simulink model "Copy_2_of_simulation"  (R2026b)
settings: Solver=ode23s  StopTime=T_sim  MaxStep=1e-3  MinStep=1e-7  RelTol=1e-5
InitFcn:
  | run param_file_2.m
values from neighbouring files (symbols this model uses):
  param = struct()    [param_file.m]    (also in param_file_2.m)
(part 2 of 2)

== matlab function Copy_2_of_simulation/MATLAB Function3 ==
  settings: updateMethod=DISCRETE  sampleTime=1e-5
  data: Pdes input; param parameter; PX input; open_PRV output; open_SSV output; PRV_position input; SSV_position input; omega input
% function [open_PRV, open_SSV] = fcn(Pdes, PX, param)
% 
% % Pressure margin for valve closure
% pressure_margin = 0.5e6;  % 0.5 MPa
% 
% if Pdes == param.P_H
% 
%     open_PRV = 1;
% 
%     % Only compress if below the high rail
%     if PX < param.P_H - pressure_margin
%         open_SSV = 1;
%     else
%         open_SSV = 0;
%     end
% 
% else
% 
%     open_PRV = -1;
% 
%     % Only decompress if above the medium rail
%     if PX > param.P_M + pressure_margin
%         open_SSV = -1;
%     else
%         open_SSV = 0;
%     end
% 
% end
% 
% end
function [open_PRV, open_SSV] = fcn(Pdes, param, PX, ...
    PRV_position, SSV_position, omega)

persistent phase switch_number current_rail

HOLD        = uint8(1);
CAPTURE     = uint8(2);
USE_ENERGY  = uint8(3);
SELECT_RAIL = uint8(4);

if isempty(phase)
    phase = HOLD;
    switch_number = uint8(1);
    current_rail = -1;          % Start on medium
end

pressure_tol = 1e4;             % Pa, 0.1 bar
spool_ready = 0.95;
ssv_center_band = 0.02;

% Each switch goes to the opposite rail.
target_rail = -current_rail;
if target_rail == 1
    target_pressure = param.P_H;
else
    target_pressure = param.P_M;
end

% Upward switch: ready when PX >= P_H - pressure_tol.
% Downward switch: ready when PX <= P_M + pressure_tol.
pressure_ready = target_rail * (target_pressure - PX) <= pressure_tol;
prv_ready = target_rail * PRV_position >= spool_ready;
switch_complete = false;

switch phase
    % case HOLD
    %     if switch_number <= 5 && Pdes == target_pressure && ...
    %             abs(SSV_position) <= ssv_center_band
    %         if switch_number <= 3
    %             phase = CAPTURE;
    %         else
    %             phase = USE_ENERGY;
    %         end
    %     end
    case HOLD
        if switch_number <= 3 && Pdes == target_pressure && ...
                abs(SSV_position) <= ssv_center_band
            if switch_number <= 2
                phase = CAPTURE;
            else
                phase = USE_ENERGY;
            end
        end

    case CAPTURE
        % The new rail is selected while the SSV routes flow through
        % the motor. Center the SSV once the transition is complete.
        if prv_ready && pressure_ready
            switch_complete = true;
        end

    case USE_ENERGY
        % Keep the previous rail selected while the shaft drives the pump.
        % Hand off at target pressure, or if the shaft runs out of speed.
        if pressure_ready || omega <= 0
            phase = SELECT_RAIL;
        end

    case SELECT_RAIL
        % Keep the SSV shifted while the PRV travels to the new rail.
        if prv_ready
            switch_complete = true;
        end
end

if switch_complete
    current_rail = target_rail;
    switch_number = switch_number + uint8(1);
    phase = HOLD;
end

% In HOLD, the selected rail stays connected and the SSV centers.
open_PRV = current_rail;
open_SSV = 0;

switch phase
    case {CAPTURE, SELECT_RAIL}
        open_PRV = target_rail;
        open_SSV = target_rail;

    case USE_ENERGY
        open_PRV = current_rail;
        open_SSV = target_rail;
end
end
%%
% function [open_PRV, open_SSV] = fcn(Pdes, clock_time, param)
% 
% t = clock_time(1);      % Simulation time [s]
% t_select_high = 0.244;  % Command PRV to high [s]
% t_center_SSV  = 0.251;  % Command SSV to center [s]
% 
% if Pdes ~= param.P_H
%     % Medium requested: select medium and center the SSV.
%     open_PRV = -1;
%     open_SSV =  0;
% 
% elseif t < t_select_high
%     % High requested: pump from medium into the chamber.
%     open_PRV = -1;
%     open_SSV =  1;
% 
% elseif t < t_center_SSV
%     % Select high while keeping the pump connected.
%     open_PRV =  1;
%     open_SSV =  1;
% 
% else
%     % Hold high and let the shaft coast.
%     open_PRV =  1;
%     open_SSV =  0;
% end
% 
% end
%%
% function [open_PRV, open_SSV] = fcn(Pdes, param, PX, ...
%     PRV_position, SSV_position, omega)
% 
% persistent stage
% 
% if isempty(stage)
%     stage = uint8(1);
% end
% 
% switch stage
%     case 1  % Hold medium until high is requested
%         if Pdes == param.P_H
%             stage = uint8(2);
%         end
% 
%     case 2  % Pump from medium into the chamber using shaft kinetic energy
%         if PX >= param.P_H
%             stage = uint8(3);
%         end
% 
%     case 3  % Wait until the PRV has physically moved to high
%         if PRV_position >= 0.95
%             stage = uint8(4);
%         end
% end
% 
% switch stage
%     case 1
%         open_PRV = -1;
%         open_SSV =  0;
%     case 2
%         open_PRV = -1;
%         open_SSV =  1;
%     case 3
%         open_PRV =  1;
%         open_SSV =  1;
%     otherwise  % Hold high for the rest of the run
%         open_PRV =  1;
%         open_SSV =  0;
% end
% end
%% New
% function [open_PRV, open_SSV] = fcn(Pdes, param, PX, ...
%     PRV_position, SSV_position, omega)
% % PRV: +1 = high rail, -1 = medium rail
% % SSV:  0 = direct rail-to-chamber connection
% %      +1 = rail to motor P, chamber to motor T
% %      -1 = chamber to motor P, rail to motor T
% 
% persistent stage
% 
% HOLD_MEDIUM    = uint8(1);
% CHARGE_TO_HIGH = uint8(2);
% HOLD_HIGH      = uint8(3);
% RETURN_TO_HIGH = uint8(4);
% SELECT_MEDIUM  = uint8(5);
% 
% if isempty(stage)
%     stage = HOLD_MEDIUM;
% end
% 
% medium_switch_margin = 0.1e6;  % Pa above the medium rail
% 
% pressure_tol = 1e4;   % Pa, same as the existing relay's 0.1 bar tolerance
% spool_ready  = 0.95;  % 95% of normalized PRV travel
% 
% % Advance the sequence using chamber pressure and actual valve position.
% switch stage
%     case HOLD_MEDIUM
%         if Pdes == param.P_H
%             stage = CHARGE_TO_HIGH;
%         end
% 
%     case CHARGE_TO_HIGH
%         if PX >= param.P_H - pressure_tol && PRV_position >= spool_ready
%             stage = HOLD_HIGH;
%         end
% 
%     case HOLD_HIGH
%         if Pdes == param.P_M
%             stage = RETURN_TO_HIGH;
%         end
% 
%     % case RETURN_TO_HIGH
%     %     % The shaft starts recovery spinning in the positive direction.
%     %     % At the first zero crossing, command the PRV to medium.
%     %     if omega <= 0
%     %         stage = SELECT_MEDIUM;
%     %     end
% 
%     case RETURN_TO_HIGH
%         if PX <= param.P_M + medium_switch_margin
%             stage = SELECT_MEDIUM;
%         end
% 
%     case SELECT_MEDIUM
%         % Keep the SSV shifted until the PRV has physically moved to medium.
%         if PRV_position <= -spool_ready
%             stage = HOLD_MEDIUM;
%         end
% end
% 
% % Issue the valve commands for the current stage.
% switch stage
%     case HOLD_MEDIUM
%         open_PRV = -1;
%         open_SSV =  0;
% 
%     case CHARGE_TO_HIGH
%         open_PRV =  1;
%         open_SSV =  1;
% 
%     case HOLD_HIGH
%         open_PRV =  1;
%         open_SSV =  0;
% 
%     case RETURN_TO_HIGH
%         open_PRV =  1;
%         open_SSV = -1;
% 
%     case SELECT_MEDIUM
%         open_PRV = -1;
%         open_SSV = -1;
% 
%     otherwise
%         open_PRV = -1;
%         open_SSV =  0;
% end
% end

%% Old
% function [open_PRV, open_SSV] = fcn(Pdes, param, PX, ...
%     PRV_position, SSV_position, omega)
% 
% persistent stage
% 
% HOLD_MEDIUM         = uint8(1);
% CHARGE_TO_HIGH      = uint8(2);
% HOLD_HIGH           = uint8(3);
% DISCHARGE_TO_MEDIUM = uint8(4);
% 
% if isempty(stage)
%     stage = HOLD_MEDIUM;
% end
% 
% pressure_tol = 1e4;   % Pa (0.1 bar)
% spool_ready  = 0.95;  % 95% of normalized PRV travel
% 
% % Advance the switching sequence.
% switch stage
%     case HOLD_MEDIUM
%         if Pdes == param.P_H
%             stage = CHARGE_TO_HIGH;
%         end
% 
%     case CHARGE_TO_HIGH
%         if PX >= param.P_H - pressure_tol && PRV_position >= spool_ready
%             stage = HOLD_HIGH;
%         end
% 
%     case HOLD_HIGH
%         if Pdes == param.P_M
%             stage = DISCHARGE_TO_MEDIUM;
%         end
% 
%     case DISCHARGE_TO_MEDIUM
%         if abs(PX - param.P_M) <= pressure_tol && ...
%                 PRV_position <= -spool_ready
%             stage = HOLD_MEDIUM;
%         end
% end
% 
% % Set valve commands for the current stage.
% switch stage
%     case CHARGE_TO_HIGH
%         open_PRV =  1;
%         open_SSV =  1;
% 
%     case HOLD_HIGH
%         open_PRV =  1;
%         open_SSV =  0;
% 
%     case DISCHARGE_TO_MEDIUM
%         open_PRV = -1;
%         open_SSV = -1;
% 
%     otherwise  % HOLD_MEDIUM
%         open_PRV = -1;
%         open_SSV =  0;
% end
% end

%% Super new
% function [open_PRV, open_SSV] = fcn(Pdes, param, PX, ...
%     PRV_position, SSV_position, omega)
% 
% persistent phase switch_number current_rail
% 
% HOLD        = uint8(1);
% STORE       = uint8(2);
% USE_ENERGY  = uint8(3);
% SELECT_RAIL = uint8(4);
% 
% if isempty(phase)
%     phase = HOLD;
%     switch_number = uint8(1);   % Next switch in the four-switch cycle
%     current_rail = -1;          % Start on medium
% end
% 
% pressure_tol    = 1e4;    % Pa, for completing a storage switch
% spool_ready     = 0.95;
% ssv_center_band = 0.02;
% 
% recovery_margin = 0.4e6;  % Switch 3: hand off 0.4 MPa below high
% P_switch4       = 4.9e6;  % Switch 4: command medium as PX falls to 5.1 MPa
% 
% % The requested sequence alternates between the two rails.
% target_rail = -current_rail;
% if target_rail == 1
%     target_pressure = param.P_H;
% else
%     target_pressure = param.P_M;
% end
% 
% % Positive while the chamber still has pressure left to gain or lose.
% pressure_remaining = target_rail * (target_pressure - PX);
% prv_at_target = target_rail * PRV_position >= spool_ready;
% 
% switch phase
%     case HOLD
%         if Pdes == target_pressure && abs(SSV_position) <= ssv_center_band
%             if switch_number <= 2
%                 phase = STORE;
%             else
%                 phase = USE_ENERGY;
%             end
%         end
% 
%     case STORE
%         % Switches 1 and 2: the pressure difference drives the shaft.
%         if prv_at_target && pressure_remaining <= pressure_tol
%             phase = HOLD;
%         end
% 
%     case USE_ENERGY
%         if switch_number == 4
%             pressure_ready = PX <= P_switch4;
%         else
%             pressure_ready = pressure_remaining <= recovery_margin;
%         end
% 
%         if pressure_ready || omega <= 0
%             phase = SELECT_RAIL;
%         end
% 
%     case SELECT_RAIL
%         % Keep the SSV shifted until the PRV reaches the target rail.
%         if prv_at_target
%             phase = HOLD;
%         end
% end
% 
% % Count a completed switch only after the PRV reaches the new rail.
% if phase == HOLD && prv_at_target
%     current_rail = target_rail;
%     if switch_number == 4
%         switch_number = uint8(1);
%     else
%         switch_number = switch_number + uint8(1);
%     end
% end
% 
% % In HOLD, center the SSV so the shaft can coast between switches.
% open_PRV = current_rail;
% open_SSV = 0;
% 
% switch phase
%     case {STORE, SELECT_RAIL}
%         open_PRV = target_rail;
%         open_SSV = target_rail;
% 
%     case USE_ENERGY
%         open_PRV = current_rail;
%         open_SSV = target_rail;
% end
% end

%% Super super new
    % function [open_PRV, open_SSV] = fcn(Pdes, param, PX, ...
    %         PRV_position, SSV_position, omega)
    % 
    %     persistent phase switch_number current_rail
    % 
    %     HOLD        = uint8(3);
    %     STORE       = uint8(4);
    %     USE_ENERGY  = uint8(2);
    %     SELECT_RAIL = uint8(1);
    % 
    %     if isempty(phase)
    %         phase = HOLD;
    %         switch_number = uint8(1);   % Next switch in the five-switch cycle
    %         current_rail = -1;          % Start on the medium rail
    %     end
    % 
    %     pressure_tol      = 1e4;    % Pa, storage-switch completion tolerance
    %     spool_ready       = 0.95;   % PRV is within 5% of its target position
    %     ssv_center_band   = 0.02;   % SSV center deadband
    %     recovery_margin   = 0.5e6;  % Pa below high for upward recovery
    %     P_handoff_down    = 4.9e6;  % Pa, chamber pressure for downward recovery
    % 
    %     % Rail positions: +1 = high, -1 = medium.
    %     target_rail = -current_rail;
    %     if target_rail == 1
    %         target_pressure = param.P_H;
    %     else
    %         target_pressure = param.P_M;
    %     end
    % 
    %     % Positive until chamber pressure reaches the target in either direction.
    %     pressure_remaining = target_rail * (target_pressure - PX);
    %     prv_at_target = target_rail * PRV_position >= spool_ready;
    % 
    %     switch_complete = false;
    % 
    %     switch phase
    %         case HOLD
    %             if Pdes == target_pressure && abs(SSV_position) <= ssv_center_band
    %                 if switch_number <= 3
    %                     phase = STORE;
    %                 else
    %                     phase = USE_ENERGY;
    %                 end
    %             end
    % 
    %         case STORE
    %             % Switches 1-3: select the target rail and accelerate the shaft.
    %             if prv_at_target && pressure_remaining <= pressure_tol
    %                 switch_complete = true;
    %             end
    % 
    %         case USE_ENERGY
    %             % Switches 4-5: keep the starting rail selected while pumping.
    %             if target_rail == -1
    %                 % High to medium: pump chamber oil back into the high rail.
    %                 pressure_ready = PX <= P_handoff_down;
    %             else
    %                 % Medium to high: pump oil from medium into the chamber.
    %                 pressure_ready = PX >= param.P_H - recovery_margin;
    %             end
    % 
    %             if pressure_ready || omega <= 0
    %                 phase = SELECT_RAIL;
    %             end
    % 
    %         case SELECT_RAIL
    %             % Keep the SSV shifted until the PRV reaches the target rail.
    %             if prv_at_target
    %                 switch_complete = true;
    %             end
    %     end
    % 
    %     % Count each completed switch once, then command the SSV to center.
    %     if switch_complete
    %         current_rail = target_rail;
    %         phase = HOLD;
    % 
    %         if switch_number == 5
    %             switch_number = uint8(1);
    %         else
    %             switch_number = switch_number + uint8(1);
    %         end
    %     end
    % 
    %     % Default HOLD commands: stay on the selected rail and coast.
    %     open_PRV = current_rail;
    %     open_SSV = 0;
    % 
    %     switch phase
    %         case {STORE, SELECT_RAIL}
    %             open_PRV = target_rail;
    %             open_SSV = target_rail;
    % 
    %         case USE_ENERGY
    %             open_PRV = current_rail;
    %             open_SSV = target_rail;
    %     end
    % 
    % end

== matlab function Copy_2_of_simulation/MATLAB Function9 ==
  data: P input; P_initial input; Win output; param parameter
function Win = oil_comp(P,P_initial,param)

Pg = P-param.P_T;   % Gauge pressure
r = P/param.P_T;    % Pressure ratio
e = exp(Pg/param.beta); 
rv = (1./e+param.air*r.^(-1/param.gamma))/(1+param.air);      %Volume ratio

El = param.beta*(e - (1 + Pg/param.beta)) + param.P_T*(e - 1);              % Energy in liquid
Eg = P/(param.gamma - 1) .* (1 - r.^(1/param.gamma - 1));           % Energy in gas
E  = (El./e + param.air*Eg.*r.^(-1/param.gamma)) ./ ...
     (1./e + param.air*r.^(-1/param.gamma));                       % Energy in mixture
Win  = E - (1./rv - 1)*P_initial;                                 % Compressibility energy density

== matlab function Copy_2_of_simulation/MATLAB Function1 ==
  data: current input; omega input; Tau_Elec output; param parameter; Tau_Mech output; Tau_Elec_Fric output
function [Tau_Elec, Tau_Mech, Tau_Elec_Fric] = BLDC(current, omega, param)

% Limit current to stall current
I_stall = 69;
current = min(max(current, -I_stall), I_stall);

% Electromagnetic torque
Tau_Elec = param.Kt * current;

% Friction torque (viscous model)
Tau_Elec_Fric = param.B * omega;

% Mechanical torque available at shaft
Tau_Mech = Tau_Elec - Tau_Elec_Fric;

end

== matlab function Copy_2_of_simulation/MATLAB Function2 ==
  data: Ph1 input; PA input; Qh1 input; Qh1dot output; param parameter
function Qh1dot = Small_Vol_A_Hose_Dynamics(Ph1, PA, Qh1, param)

Qh1dot = ((Ph1 - PA) - param.ResistHose*Qh1)/param.InertHose;

== matlab function Copy_2_of_simulation/Electric Torque Controller1 ==
  data: Control_Signal input; Kp input; omega input; T_elec output; start_final_velocity input; T_elec_max input; param parameter
% function T_elec  = fcn(Control_Signal, Kp, omega, start_final_velocity, T_elec_max, param)
% 
% if Control_Signal == 1 
% 
%     if omega < start_final_velocity
%         omega_error = omega -start_final_velocity;
%         T_elec = - (Kp*omega_error);
%     else
%         T_elec = -T_elec_max;
%     end
% 
% else
%     if omega >= param.max_speed-0.01
%         omega_error = omega - param.max_speed;
%         T_elec = -(Kp*omega_error);
%     else
%         T_elec = T_elec_max;
%     end
% 
% end

function T_elec = fcn(Control_Signal, Kp, omega, ...
    start_final_velocity, T_elec_max, param)

if Control_Signal == 1
    target_speed = start_final_velocity;
else
    target_speed = param.max_speed;
end

omega_error = omega - target_speed;

T_elec = -Kp * omega_error;

% Saturate torque
T_elec = min(max(T_elec, -T_elec_max), T_elec_max);

end

== matlab function Copy_2_of_simulation/Small Volume A1 ==
  data: Qh1 input; QA input; PAdot output; param parameter
function PAdot = Small_Vol_A(Qh1,QA, param)

PAdot = (param.beta/param.VA_0)*(Qh1-QA);

== matlab function Copy_2_of_simulation/MATLAB Function4 ==
  data: Ph1 input; PA input; Qh1 output; param parameter
function Qh1 = Small_Vol_A_Hose_Dynamics(Ph1, PA, param)

Qh1 = (Ph1 - PA)/param.ResistHose;

== matlab function Copy_2_of_simulation/Small Volume A2 ==
  data: Q1 input; PAdot output; QA input; beta_mix input; param parameter
function PAdot = Small_Vol_A(Q1,QA, beta_mix, param)

PAdot = (beta_mix/param.VA_0)*(Q1-QA);

== matlab function Copy_2_of_simulation/MATLAB Function5 ==
  data: P input; P_initial input; beta_mix_A output; param parameter; WA output
function [beta_mix_A, WA] = oil_comp(P,P_initial,param)

Pg = P-param.P_T;   % Gauge pressure
r = P/param.P_T;    % Pressure ratio
e = exp(Pg/param.beta); 
rv = (1./e+param.air*r.^(-1/param.gamma))/(1+param.air);      %Volume ratio

beta_mix_A = rv*(1+param.air)/(1/(e*param.beta)+...
           param.air/(param.gamma*param.P_T*r^(1/param.gamma+1)));

El = param.beta*(e - (1 + Pg/param.beta)) + param.P_T*(e - 1);              % Energy in liquid
Eg = P/(param.gamma - 1) .* (1 - r.^(1/param.gamma - 1));           % Energy in gas
E  = (El./e + param.air*Eg.*r.^(-1/param.gamma)) ./ ...
     (1./e + param.air*r.^(-1/param.gamma));                       % Energy in mixture
WA  = E - (1./rv - 1)*P_initial;                                 % Compressibility energy density

== matlab function Copy_2_of_simulation/MATLAB Function6 ==
  data: P input; P_initial input; beta_mix output; param parameter; WP output
function [beta_mix, WP] = oil_comp(P,P_initial,param)

%Ph=7e6, P0=1e5
Pg = P-param.P_T;   % Gauge pressure
r = P/param.P_T;    % Pressure ratio
e = exp(Pg/param.beta); 
rv = (1./e+param.air*r.^(-1/param.gamma))/(1+param.air);      %Volume ratio

beta_mix = rv*(1+param.air)/(1/(e*param.beta)+...
           param.air/(param.gamma*param.P_T*r^(1/param.gamma+1)));

El = param.beta*(e - (1 + Pg/param.beta)) + param.P_T*(e - 1);              % Energy in liquid
Eg = P/(param.gamma - 1) .* (1 - r.^(1/param.gamma - 1));           % Energy in gas
E  = (El./e + param.air*Eg.*r.^(-1/param.gamma)) ./ ...
     (1./e + param.air*r.^(-1/param.gamma));                       % Energy in mixture
WP  = E - (1./rv - 1)*P_initial;                                 % Compressibility energy density

== matlab function Copy_2_of_simulation/Small Volume A ==
  data: Q1 input; Ph1dot output; Qh1 input; param parameter
function Ph1dot = Small_Vol_A(Q1,Qh1, param)

Ph1dot = (param.beta/param.VA_0)*(Q1-Qh1);

== matlab function Copy_2_of_simulation/MATLAB Function7 ==
  data: P input; P_initial input; beta_mix output; param parameter; WT output
function [beta_mix, WT] = oil_comp(P,P_initial,param)

%Ph=7e6, P0=1e5
Pg = P-param.P_T;   % Gauge pressure
r = P/param.P_T;    % Pressure ratio
e = exp(Pg/param.beta); 
rv = (1./e+param.air*r.^(-1/param.gamma))/(1+param.air);      %Volume ratio

beta_mix = rv*(1+param.air)/(1/(e*param.beta)+...
           param.air/(param.gamma*param.P_T*r^(1/param.gamma+1)));


El = param.beta*(e - (1 + Pg/param.beta)) + param.P_T*(e - 1);              % Energy in liquid
Eg = P/(param.gamma - 1) .* (1 - r.^(1/param.gamma - 1));           % Energy in gas
E  = (El./e + param.air*Eg.*r.^(-1/param.gamma)) ./ ...
     (1./e + param.air*r.^(-1/param.gamma));                       % Energy in mixture
WT  = E - (1./rv - 1)*P_initial;                                 % Compressibility energy density

== matlab function Copy_2_of_simulation/MATLAB Function8 ==
  data: P input; P_initial input; beta_mix output; param parameter; WX output
function [beta_mix, WX] = oil_comp(P,P_initial,param)

%Ph=7e6, P0=1e5
Pg = P-param.P_T;   % Gauge pressure
r = P/param.P_T;    % Pressure ratio
e = exp(Pg/param.beta); 
rv = (1./e+param.air*r.^(-1/param.gamma))/(1+param.air);      %Volume ratio

beta_mix = rv*(1+param.air)/(1/(e*param.beta)+...
           param.air/(param.gamma*param.P_T*r^(1/param.gamma+1)));

El = param.beta*(e - (1 + Pg/param.beta)) + param.P_T*(e - 1);              % Energy in liquid
Eg = P/(param.gamma - 1) .* (1 - r.^(1/param.gamma - 1));           % Energy in gas
E  = (El./e + param.air*Eg.*r.^(-1/param.gamma)) ./ ...
     (1./e + param.air*r.^(-1/param.gamma));                       % Energy in mixture
WX  = E - (1./rv - 1)*P_initial;                                 % Compressibility energy density

== matlab function Copy_2_of_simulation/MATLAB Function ==
  data: beta_mix input; Stored_Power output; Pdot input; P input; Volume input
function Stored_Power = fcn(beta_mix, Pdot, P, Volume)

Stored_Power = P*(Volume/beta_mix)*Pdot;

== matlab function Copy_2_of_simulation/MATLAB Function10 ==
  data: beta_mix input; Stored_Power output; Pdot input; P input; Volume input
function Stored_Power = fcn(beta_mix, Pdot, P, Volume)

Stored_Power = P*(Volume/beta_mix)*Pdot;

== matlab function Copy_2_of_simulation/MATLAB Function11 ==
  data: beta_mix input; Stored_Power output; Pdot input; P input; Volume input
function Stored_Power = fcn(beta_mix, Pdot, P, Volume)

Stored_Power = P*(Volume/beta_mix)*Pdot;

== matlab function Copy_2_of_simulation/MATLAB Function12 ==
  data: clock_time input; Pdes output; param parameter
function Pdes = fcn(clock_time, param)

t = clock_time(1);

if t < 0.20
    Pdes = param.P_M;
elseif t < 0.75
    Pdes = param.P_H;   % Switch 1: medium to high
elseif t < 1.30
    Pdes = param.P_M;   % Switch 2: high to medium
else
    Pdes = param.P_H;   % Switch 3: medium to high
end

end

% function Pdes = fcn(clock_time, param)
% 
% t = clock_time(1);
% 
% if (t >= 0.20 && t < 0.75) || ...
%         (t >= 1.30 && t < 1.85) || ...
%         t >= 2.40
%     Pdes = param.P_H;
% else
%     Pdes = param.P_M;
% end
% 
% end

% t = clock_time(1);
% 
% if (t >= 0.20 && t < 0.75) || ...
%         (t >= 1.30 && t < 1.85) || ...
%         t >= 2.40
%     Pdes = param.P_H;
% else
%     Pdes = param.P_M;
% end
% 
% end

% function Pdes = fcn(clock_time, param)
% 
% if (clock_time >= 0.20 && clock_time < 0.75) || ...
%         (clock_time >= 1.30 && clock_time < 1.85)
%     Pdes = param.P_H;
% else
%     Pdes = param.P_M;
% end
% 
% end

== matlab function Copy_2_of_simulation/Experimental Friction Model ==
  data: pressure input; friction output; speed input
function friction  = friction_model(pressure, speed)

C = [-2.7371712380878151e-20 -1.012140531055926e-17 1.362680380791501e-14 2.5017160289203132e-12;
    7.8175012770957013e-17 6.5819426994446848e-14 -5.7218700361030071e-11 -2.6554187394929447e-08;
    -3.0602563559828119e-14 -2.3014653747973892e-10 2.0537443634696756e-07 0.00011211247665566631;
    8.9217552784699898e-12 5.982060290372595e-08 7.3192331395694632e-05 0.083988065486528374];

p = [pressure^3; pressure^2; pressure; 1];
w = [speed^3; speed^2; speed; 1];

friction = sum((C * p) .* w);
end

== matlab function Copy_2_of_simulation/MATLAB Function13 ==
  data: current_in input; current output; elec_motor input
function current = fcn(current_in, elec_motor)

if elec_motor == 1
    current = current_in;
elseif elec_motor == 0
    current = 0;
else
    current = 0;
end

== matlab function Copy_2_of_simulation/MATLAB Function14 ==
  data: inertia output; elec_motor input; param parameter
function inertia = fcn(elec_motor, param)

if elec_motor == 1
    inertia = (param.J_hyd+param.J_elec);
elseif elec_motor == 0
    inertia = param.J_hyd;
else
    inertia = 0;
end

== matlab function Copy_2_of_simulation/MATLAB Function15 ==
  data: Q_PA input; Q_AT input; rail_power output; PA input; PRV_loss_power output; param parameter
% function [rail_power, PRV_loss_power] = fcn(Q1, PA, PRV_position, param)
% 
% if PRV_position < -param.valve_buffer
%     P_rail = param.P_M;
% elseif PRV_position > param.valve_buffer
%     P_rail = param.P_H;
% else
%     % Both rail passages are closed.
%     rail_power = 0;
%     PRV_loss_power = 0;
%     return
% end
% 
% rail_power     = P_rail * Q1;         % Signed power supplied by the rail [W]
% PRV_loss_power = (P_rail - PA) * Q1;  % Power dissipated across the PRV [W]
% end

function [rail_power, PRV_loss_power] = fcn(Q_PA, Q_AT, PA, param)

% Both flows are positive from their respective rail toward port A.
rail_power = param.P_H * Q_PA + param.P_M * Q_AT;

PRV_loss_power = (param.P_H - PA) * Q_PA + ...
    (param.P_M - PA) * Q_AT;
end

== matlab function Copy_2_of_simulation/Pressure Rail Valve ==
  data: P input; T input; Q_PA output; Q_AT output; PA input; spool_position input; param parameter
% function [Q_PA, Q_AT] = RailValve(P, T, PA, spool_position, param)
% 
% db = param.valve_buffer;
% 
% spool_position = max(-1, min(1, spool_position));
% 
% if abs(spool_position) <= db
%     f = 0;
% else
%     f = (abs(spool_position) - db) / (1 - db);
%     f = max(0, min(1, f));
% end
% 
% A_PA = 0;
% A_AT = 0;
% 
% if spool_position > db
%     A_PA = param.max_Avt * f;
% elseif spool_position < -db
%     A_AT = param.max_Avt * f;
% end
% 
% Q_PA = param.Cd * A_PA * sqrt(2/param.rho) * sqrt(abs(P-PA)) * sign(P-PA);
% Q_AT = param.Cd * A_AT * sqrt(2/param.rho) * sqrt(abs(PA-T)) * sign(T-PA);
% 
% end

function [Q_PA, Q_AT] = RailValve(P, T, PA, spool_position, param)

db = param.valve_buffer;
dp_smooth = param.dp_smooth;   % Pa: smoothing scale (0.01 bar)

spool_position = max(-1, min(1, spool_position));

if abs(spool_position) <= db
    f = 0;
else
    f = (abs(spool_position) - db) / (1 - db);
    f = max(0, min(1, f));
end

A_PA = 0;
A_AT = 0;

if spool_position > db
    A_PA = param.max_Avt * f;
elseif spool_position < -db
    A_AT = param.max_Avt * f;
end

% Positive flow is from each rail toward port A.
dP_PA = P - PA;
dP_AT = T - PA;

% Smoothed signed square-root pressure relationship.
Q_PA = param.Cd * A_PA * sqrt(2/param.rho) * ...
    dP_PA / (dP_PA^2 + dp_smooth^2)^0.25;

Q_AT = param.Cd * A_AT * sqrt(2/param.rho) * ...
    dP_AT / (dP_AT^2 + dp_smooth^2)^0.25;

end

== matlab function Copy_2_of_simulation/Electric Torque Controller2 ==
  data: Control_Signal input; Kp input; omega input; T_elec output; start_final_velocity input; T_elec_max input; param parameter
% function T_elec  = fcn(Control_Signal, Kp, omega, start_final_velocity, T_elec_max, param)
% 
% if Control_Signal == 1 
% 
%     if omega < start_final_velocity
%         omega_error = omega -start_final_velocity;
%         T_elec = - (Kp*omega_error);
%     else
%         T_elec = -T_elec_max;
%     end
% 
% else
%     if omega >= param.max_speed-0.01
%         omega_error = omega - param.max_speed;
%         T_elec = -(Kp*omega_error);
%     else
%         T_elec = T_elec_max;
%     end
% 
% end

function T_elec = fcn(Control_Signal, Kp, omega, ...
    start_final_velocity, T_elec_max, param)

if Control_Signal == 1
    target_speed = start_final_velocity;
else
    target_speed = param.max_speed;
end

omega_error = omega - target_speed;

T_elec = -Kp * omega_error;

% Saturate torque
T_elec = min(max(T_elec, -T_elec_max), T_elec_max);

end

== matlab function Copy_2_of_simulation/MATLAB Function16 ==
  data: clock_time input; Pdes output; param parameter
function Pdes = fcn(clock_time, param)

if clock_time > 0.2 && clock_time < 0.75
    Pdes = param.P_H;
else
    Pdes = param.P_M;
end

== matlab function Copy_2_of_simulation/MATLAB Function17 ==
  data: Pdes input; PX input; open_PRV output; open_SSV output; param parameter
% function [open_PRV, open_SSV] = fcn(Pdes, param, Control_signal)
% 
% if Pdes == param.P_H && Control_signal == 0
%     open_PRV = 1;
%     open_SSV = 1;
% 
% elseif Pdes == param.P_M && Control_signal == 0
%     open_PRV = -1;
%     open_SSV = -1;
% 
% elseif Pdes == param.P_H && Control_signal > 0
%     open_PRV = 1;
%     open_SSV = 0;
% 
% elseif Pdes == param.P_M && Control_signal > 0
%     open_PRV = -1;
%     open_SSV = 0;
% 
% else
%     open_PRV = 0;
%     open_SSV = 0;
% end


function [open_PRV, open_SSV] = fcn(Pdes, PX, param)

% Pressure margin for valve closure
pressure_margin = 0.5e6;  % 0.5 MPa

if Pdes == param.P_H

    open_PRV = 1;

    % Only compress if below the high rail
    if PX < param.P_H - pressure_margin
        open_SSV = 1;
    else
        open_SSV = 0;
    end

else

    open_PRV = -1;

    % Only decompress if above the medium rail
    if PX > param.P_M + pressure_margin
        open_SSV = -1;
    else
        open_SSV = 0;
    end

end

end

== matlab function Copy_2_of_simulation/Soft-switch Valve ==
  data: spool_position input; Q_P output; PP input; PA input; PB input; PT input; Q_A output; Q_B output; Q_T output; param parameter; SSV_Power_throttle output; WA input; WP input; WB input; WT input; SSV_Power_throttle_HE output
% function [Q_P, Q_A, Q_B, Q_T, SSV_Power_throttle, SSV_Power_throttle_HE] = SSV(spool_position, PP, PA, PB, PT, param, WA, WP, WB, WT)
% 
% db = 0.02; % spool deadband around zero (fraction of full stroke)
% 
% spool_position = max(-1, min(1, spool_position));
% 
% if abs(spool_position) <= db
%     f = 0;
% else
%     f = (abs(spool_position) - db) / (1 - db);
%     f = max(0, min(1, f));
% end
% 
% A_PA = 0; A_PB = 0; A_AT = 0; A_BT = 0; A_PT = 0; A_AB = 0;
% 
% if abs(spool_position) <= db
%     A_PT = param.max_Avt;
%     A_AB = param.max_Avt;
% elseif spool_position > 0
%     A_PA = param.max_Avt * f;
%     A_BT = param.max_Avt * f;
% elseif spool_position < 0
%     A_PB = param.max_Avt * f;
%     A_AT = param.max_Avt * f;
% end
% 
% Q_PA = param.Cd*A_PA*sign(PP-PA)*sqrt((2/param.rho)*abs(PP-PA));
% Q_PB = param.Cd*A_PB*sign(PP-PB)*sqrt((2/param.rho)*abs(PP-PB));
% Q_AT = param.Cd*A_AT*sign(PA-PT)*sqrt((2/param.rho)*abs(PA-PT));
% Q_BT = param.Cd*A_BT*sign(PB-PT)*sqrt((2/param.rho)*abs(PB-PT));
% Q_PT = param.Cd*A_PT*sign(PP-PT)*sqrt((2/param.rho)*abs(PP-PT));
% Q_AB = param.Cd*A_AB*sign(PA-PB)*sqrt((2/param.rho)*abs(PA-PB));
% 
% Q_P = -(Q_PA + Q_PB + Q_PT);
% Q_A =  Q_AT + Q_AB - Q_PA;
% Q_B =  Q_BT - Q_AB - Q_PB;
% Q_T =  -Q_PT - Q_AT - Q_BT;
% 
% Q_B = -Q_B;
% 
% PPg = PP - param.P_T;
% PAg = PA - param.P_T;
% PBg = PB - param.P_T;
% PTg = PT - param.P_T;
% 
% SSV_Power_throttle_HE = ...
%     abs(Q_PA)*abs((WP+PPg)-(WA+PAg)) + ...
%     abs(Q_PB)*abs((WP+PPg)-(WB+PBg)) + ...
%     abs(Q_AT)*abs((WA+PAg)-(WT+PTg)) + ...
%     abs(Q_BT)*abs((WB+PBg)-(WT+PTg)) + ...
%     abs(Q_PT)*abs((WP+PPg)-(WT+PTg)) + ...
%     abs(Q_AB)*abs((WA+PAg)-(WB+PBg));
% 
% SSV_Power_throttle = ...
%     abs(Q_PA)*abs(PP-PA) + ...
%     abs(Q_PB)*abs(PP-PB) + ...
%     abs(Q_AT)*abs(PA-PT) + ...
%     abs(Q_BT)*abs(PB-PT) + ...
%     abs(Q_PT)*abs(PP-PT) + ...
%     abs(Q_AB)*abs(PA-PB);
% 
% end

function [Q_P, Q_A, Q_B, Q_T, SSV_Power_throttle, ...
    SSV_Power_throttle_HE] = SSV(spool_position, ...
    PP, PA, PB, PT, param, WA, WP, WB, WT)

db = 0.02;        % Spool deadband
dp_smooth = param.dp_smooth;  % Pa: smoothing scale (0.01 bar)

spool_position = max(-1, min(1, spool_position));

if abs(spool_position) <= db
    f = 0;
else
    f = (abs(spool_position) - db) / (1 - db);
    f = max(0, min(1, f));
end

A_PA = 0;
A_PB = 0;
A_AT = 0;
A_BT = 0;
A_PT = 0;
A_AB = 0;

if abs(spool_position) <= db
    A_PT = param.max_Avt;
    A_AB = param.max_Avt;
elseif spool_position > 0
    A_PA = param.max_Avt * f;
    A_BT = param.max_Avt * f;
elseif spool_position < 0
    A_PB = param.max_Avt * f;
    A_AT = param.max_Avt * f;
end

% Signed pressure differences
dP_PA = PP - PA;
dP_PB = PP - PB;
dP_AT = PA - PT;
dP_BT = PB - PT;
dP_PT = PP - PT;
dP_AB = PA - PB;

% Smoothed orifice flows
C = param.Cd * sqrt(2/param.rho);

Q_PA = C*A_PA*dP_PA / (dP_PA^2 + dp_smooth^2)^0.25;
Q_PB = C*A_PB*dP_PB / (dP_PB^2 + dp_smooth^2)^0.25;
Q_AT = C*A_AT*dP_AT / (dP_AT^2 + dp_smooth^2)^0.25;
Q_BT = C*A_BT*dP_BT / (dP_BT^2 + dp_smooth^2)^0.25;
Q_PT = C*A_PT*dP_PT / (dP_PT^2 + dp_smooth^2)^0.25;
Q_AB = C*A_AB*dP_AB / (dP_AB^2 + dp_smooth^2)^0.25;

% Port flows: retain existing sign conventions
Q_P = -(Q_PA + Q_PB + Q_PT);
Q_A =  Q_AT + Q_AB - Q_PA;
Q_B =  Q_BT - Q_AB - Q_PB;
Q_T = -Q_PT - Q_AT - Q_BT;

Q_B = -Q_B;

% Gauge pressures
PPg = PP - param.P_T;
PAg = PA - param.P_T;
PBg = PB - param.P_T;
PTg = PT - param.P_T;

% Hydraulic-effort calculation: retain existing definition
SSV_Power_throttle_HE = ...
    abs(Q_PA)*abs((WP+PPg)-(WA+PAg)) + ...
    abs(Q_PB)*abs((WP+PPg)-(WB+PBg)) + ...
    abs(Q_AT)*abs((WA+PAg)-(WT+PTg)) + ...
    abs(Q_BT)*abs((WB+PBg)-(WT+PTg)) + ...
    abs(Q_PT)*abs((WP+PPg)-(WT+PTg)) + ...
    abs(Q_AB)*abs((WA+PAg)-(WB+PBg));

% Throttling power calculated using the smoothed flows
SSV_Power_throttle = ...
    abs(Q_PA)*abs(dP_PA) + ...
    abs(Q_PB)*abs(dP_PB) + ...
    abs(Q_AT)*abs(dP_AT) + ...
    abs(Q_BT)*abs(dP_BT) + ...
    abs(Q_PT)*abs(dP_PT) + ...
    abs(Q_AB)*abs(dP_AB);

end

== matlab function Copy_2_of_simulation/Small Volume P ==
  data: QP input; PPdot output; Qpump input; param parameter; beta_mix input
function PPdot = Small_Vol_P(QP,Qpump, param, beta_mix)

PPdot = (beta_mix/param.VP_0)*(QP-Qpump);

== matlab function Copy_2_of_simulation/Hydraulic Motor ==
  data: Qpump output; Qleak output; omega input; PT input; PP input; fric input; param parameter; DeltaP output; Tau_Pump output; Tau_Fric output
function [Qpump, Qleak, DeltaP, Tau_Pump, Tau_Fric] = Hyd_Motor(omega, PT, PP, fric, param)

    DeltaP = PP - PT;

    Tau_Ideal = (param.D/(2*pi)) * DeltaP;
    
    % Pump friction model
    if fric == 1
        Tau_fr_nom = ((1 - param.eta_m_nom)/param.eta_m_nom) ...
                      * (param.D/(2*pi)) * param.dp_nom;
        
        k = (Tau_fr_nom - param.tau0) / param.dp_nom;
        
        omega_nom_rad = 2*pi*param.omega_nom/60;
        
        s = tanh(4*omega/(5e-5*omega_nom_rad));
        
        Tau_Fric = (param.tau0 + k*abs(DeltaP)) * s;
    else
        Tau_Fric = 0;
    end

    Tau_Pump = Tau_Ideal - Tau_Fric;

    % Analytical leakage model (Simscape-equivalent)
    
    % Parameters
    D     = param.D;          
    eta_v = param.eta_v_nom;  % nominal volumetric efficiency
    omega_nom = param.omega_nom;      % [rad/s]
    DeltaP_nom = param.dp_nom;    % [Pa]
    rho   = param.rho;        % [kg/m^3]
    
    % Hagen–Poiseuille coefficient
    K = (D/(2*pi))*omega_nom*(1 - eta_v)/DeltaP_nom;
    
    % Mass leakage flow
    m_dot_leak = K * rho * DeltaP;
    
    % Convert to volumetric leakage
    Qleak = m_dot_leak / rho;
    
    % Ideal displacement flow
    Qideal = (D/(2*pi)) * omega;
    
    % Net flow (same convention as Simscape)
    Qpump = Qideal + Qleak;
end

== matlab function Copy_2_of_simulation/Small Volume T ==
  data: QT input; PTdot output; Qpump input; param parameter; beta_mix input
function PTdot = Small_Vol_T(QT,Qpump,param, beta_mix)

PTdot = (beta_mix/param.VT_0)*(Qpump-QT);

== matlab function Copy_2_of_simulation/Main Chamber ==
  data: QB input; PXdot output; param parameter; beta_mix input
function PXdot = Main_Chamber(QB, param, beta_mix)

PXdot = (beta_mix/param.V1_0)*(QB);
